simulink model "SystemStartupActivity"  (R2024a)
settings: Solver=VariableStepAuto  StartTime=0.0  StopTime=10.0  RelTol=1e-3
settings Model: Creator=joshkahn  LastModifiedBy=joshkahn

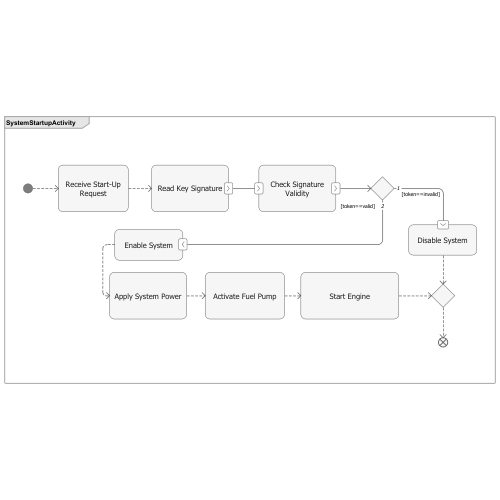
[thumbnail: Simulink's stored preview of the top-level diagram]
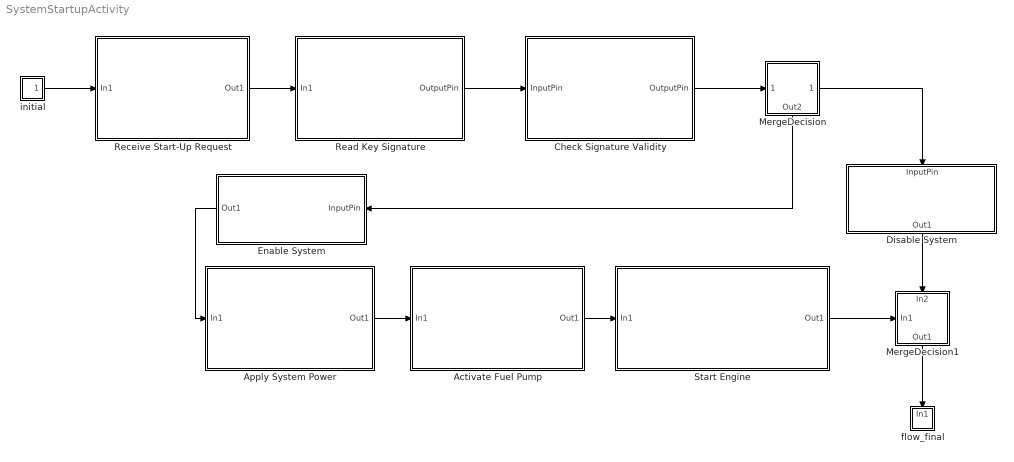
== system SystemStartupActivity ==
  Activate Fuel Pump : Subsystem
      settings: CopyFcn=set_param(gcbh,'LinkStatus','none');
  Apply System Power : Subsystem
      settings: CopyFcn=set_param(gcbh,'LinkStatus','none');
  Check Signature Validity : Subsystem
      settings: CopyFcn=set_param(gcbh,'LinkStatus','none');
  Disable System : Subsystem
      settings: CopyFcn=set_param(gcbh,'LinkStatus','none');  PortSchema="{\"entries\":[{\"content\":{\"sides\":[{\"content\":{},\"type\":\"ConnectorPlacement.EquallySpacedRectSide\",\"uuid\":\"85fc344b-9b95-4298-8a50-efffe9d97adb\"},{\"content\":{\"side\":\"RIGHT\"},\"type\":\"ConnectorPlacement.EquallySpacedRectSide\",\"uuid\":\"e59eb403-61b4-4d5a-9d35-239934c37bcd\"},{\"content\":{\"connectorIds\":[\"In1\"],\"side\":\"TOP\"},\"type\":\"ConnectorPlacement.EquallySpacedRectSide\",\"uuid\":\"05b08ca4-e27e-4f19-9584-67ae5adbaa3a\"},{\"content\":{\"connectorIds\":[\"Out1\"],\"side\":\"BOTTOM\"},\"type\":\"ConnectorPlacement.EquallySpacedRectSide\",\"uuid\":\"884202e7-807c-41e2-a007-b07e7ac04fc2\"}]},\"type\":\"ConnectorPlacement.EquallySpacedConnector\",\"uuid\":\"e4a982cb-7802-4b33-8ec4-bde570d0077e\"}],\"packageUris\":[\"http://schema.mathworks.com/mf0/Connector/R2020b\"],\"version\":\"1.0\"}"
  Enable System : Subsystem
      settings: CopyFcn=set_param(gcbh,'LinkStatus','none');  PortSchema="{\"entries\":[{\"content\":{\"sides\":[{\"content\":{\"connectorIds\":[\"Out1\"]},\"type\":\"ConnectorPlacement.EquallySpacedRectSide\",\"uuid\":\"85fc344b-9b95-4298-8a50-efffe9d97adb\"},{\"content\":{\"connectorIds\":[\"In1\"],\"side\":\"RIGHT\"},\"type\":\"ConnectorPlacement.EquallySpacedRectSide\",\"uuid\":\"e59eb403-61b4-4d5a-9d35-239934c37bcd\"},{\"content\":{\"side\":\"TOP\"},\"type\":\"ConnectorPlacement.EquallySpacedRectSide\",\"uuid\":\"05b08ca4-e27e-4f19-9584-67ae5adbaa3a\"},{\"content\":{\"side\":\"BOTTOM\"},\"type\":\"ConnectorPlacement.EquallySpacedRectSide\",\"uuid\":\"884202e7-807c-41e2-a007-b07e7ac04fc2\"}]},\"type\":\"ConnectorPlacement.EquallySpacedConnector\",\"uuid\":\"e4a982cb-7802-4b33-8ec4-bde570d0077e\"}],\"packageUris\":[\"http://schema.mathworks.com/mf0/Connector/R2020b\"],\"version\":\"1.0\"}"
  MergeDecision : Subsystem
      settings: CopyFcn=set_param(gcbh,'LinkStatus','none');  PortSchema="{\"entries\":[{\"content\":{\"sides\":[{\"content\":{\"connectorIds\":[\"In1\"]},\"type\":\"ConnectorPlacement.EquallySpacedRectSide\",\"uuid\":\"566c0eec-a2dd-4a6d-9f53-2c009cb0427b\"},{\"content\":{\"connectorIds\":[\"Out1\"],\"side\":\"RIGHT\"},\"type\":\"ConnectorPlacement.EquallySpacedRectSide\",\"uuid\":\"1e04f943-f9f7-41b9-b1a9-f47614b7de44\"},{\"content\":{\"side\":\"TOP\"},\"type\":\"ConnectorPlacement.EquallySpacedRectSide\",\"uuid\":\"7226c155-6dd2-407f-9ff6-15220628bc2f\"},{\"content\":{\"connectorIds\":[\"Out2\"],\"side\":\"BOTTOM\"},\"type\":\"ConnectorPlacement.EquallySpacedRectSide\",\"uuid\":\"5b8beda2-57dc-4ae1-a074-ab5bb5a3d918\"}]},\"type\":\"ConnectorPlacement.EquallySpacedConnector\",\"uuid\":\"7f8ec6b0-51a3-49f4-933e-41c7d4219391\"}],\"packageUris\":[\"http://schema.mathworks.com/mf0/Connector/R2020b\"],\"version\":\"1.0\"}"
  MergeDecision1 : Subsystem
      settings: CopyFcn=set_param(gcbh,'LinkStatus','none');  PortSchema="{\"entries\":[{\"content\":{\"sides\":[{\"content\":{\"connectorIds\":[\"In1\"]},\"type\":\"ConnectorPlacement.EquallySpacedRectSide\",\"uuid\":\"566c0eec-a2dd-4a6d-9f53-2c009cb0427b\"},{\"content\":{\"side\":\"RIGHT\"},\"type\":\"ConnectorPlacement.EquallySpacedRectSide\",\"uuid\":\"1e04f943-f9f7-41b9-b1a9-f47614b7de44\"},{\"content\":{\"connectorIds\":[\"In2\"],\"side\":\"TOP\"},\"type\":\"ConnectorPlacement.EquallySpacedRectSide\",\"uuid\":\"7226c155-6dd2-407f-9ff6-15220628bc2f\"},{\"content\":{\"connectorIds\":[\"Out1\"],\"side\":\"BOTTOM\"},\"type\":\"ConnectorPlacement.EquallySpacedRectSide\",\"uuid\":\"d38e6ec2-2250-46b2-b61c-13627388fd92\"}]},\"type\":\"ConnectorPlacement.EquallySpacedConnector\",\"uuid\":\"7f8ec6b0-51a3-49f4-933e-41c7d4219391\"}],\"packageUris\":[\"http://schema.mathworks.com/mf0/Connector/R2020b\"],\"version\":\"1.0\"}"
  Read Key Signature : Subsystem
      settings: CopyFcn=set_param(gcbh,'LinkStatus','none');
  Receive Start-Up Request : Subsystem
      settings: CopyFcn=set_param(gcbh,'LinkStatus','none');
  Start Engine : Subsystem
      settings: CopyFcn=set_param(gcbh,'LinkStatus','none');
  flow_final : Subsystem
      settings: CopyFcn=set_param(gcbh,'LinkStatus','none');  PortSchema="{\"entries\":[{\"content\":{\"sides\":[{\"content\":{},\"type\":\"ConnectorPlacement.EquallySpacedRectSide\",\"uuid\":\"85fc344b-9b95-4298-8a50-efffe9d97adb\"},{\"content\":{\"side\":\"RIGHT\"},\"type\":\"ConnectorPlacement.EquallySpacedRectSide\",\"uuid\":\"e59eb403-61b4-4d5a-9d35-239934c37bcd\"},{\"content\":{\"connectorIds\":[\"In1\"],\"side\":\"TOP\"},\"type\":\"ConnectorPlacement.EquallySpacedRectSide\",\"uuid\":\"05b08ca4-e27e-4f19-9584-67ae5adbaa3a\"}]},\"type\":\"ConnectorPlacement.EquallySpacedConnector\",\"uuid\":\"e4a982cb-7802-4b33-8ec4-bde570d0077e\"}],\"packageUris\":[\"http://schema.mathworks.com/mf0/Connector/R2020b\"],\"version\":\"1.0\"}"
  initial : Subsystem
      settings: CopyFcn=set_param(gcbh,'LinkStatus','none');
  wires:
  Read Key Signature/1(OutputPin) -> Check Signature Validity/1(InputPin)
  initial/1(Out1) -> Receive Start-Up Request/1(In1)
  Receive Start-Up Request/1(Out1) -> Read Key Signature/1(In1)
  Start Engine/1(Out1) -> MergeDecision1/1(In1)
  Check Signature Validity/1(OutputPin) -> MergeDecision/1(InputPin)
  MergeDecision/1(Out1) -> Disable System/1(InputPin)
  Disable System/1(Out1) -> MergeDecision1/2(In2)
  MergeDecision/2(Out2) -> Enable System/1(InputPin)
  Enable System/1(Out1) -> Apply System Power/1(In1)
  Apply System Power/1(Out1) -> Activate Fuel Pump/1(In1)
  Activate Fuel Pump/1(Out1) -> Start Engine/1(In1)
  MergeDecision1/1(Out1) -> flow_final/1(In1)

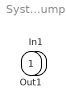
== system SystemStartupActivity/Activate Fuel Pump ==
  In1 : Inport
  Out1 : Outport

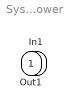
== system SystemStartupActivity/Apply System Power ==
  In1 : Inport
  Out1 : Outport

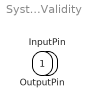
== system SystemStartupActivity/Check Signature Validity ==
  InputPin : Inport
  OutputPin : Outport  OutDataTypeStr=double  PortDimensions=1

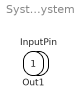
== system SystemStartupActivity/Disable System ==
  InputPin : Inport
  Out1 : Outport

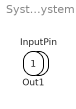
== system SystemStartupActivity/Enable System ==
  InputPin : Inport
  Out1 : Outport

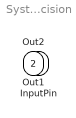
== system SystemStartupActivity/MergeDecision ==
  InputPin : Inport
  Out1 : Outport
  Out2 : Outport  Port=2

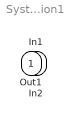
== system SystemStartupActivity/MergeDecision1 ==
  In1 : Inport
  In2 : Inport  Port=2
  Out1 : Outport

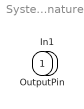
== system SystemStartupActivity/Read Key Signature ==
  In1 : Inport
  OutputPin : Outport  OutDataTypeStr=double  PortDimensions=1

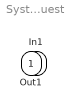
== system SystemStartupActivity/Receive Start-Up Request ==
  In1 : Inport
  Out1 : Outport

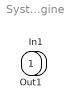
== system SystemStartupActivity/Start Engine ==
  In1 : Inport
  Out1 : Outport

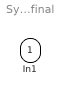
== system SystemStartupActivity/flow_final ==
  In1 : Inport

== system SystemStartupActivity/initial ==
  Out1 : Outport
